simulink model "SimulinkController"  (R2026a)
settings: Solver=VariableStepAuto
libraries: cstblocks_lti x6, simulink_extras x4
settings Model: Creator=ASUS TUF  LastModifiedBy=ASUS TUF

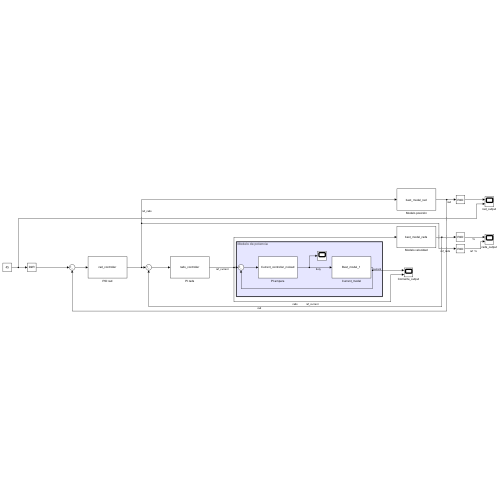
[thumbnail: Simulink's stored preview of the top-level diagram]
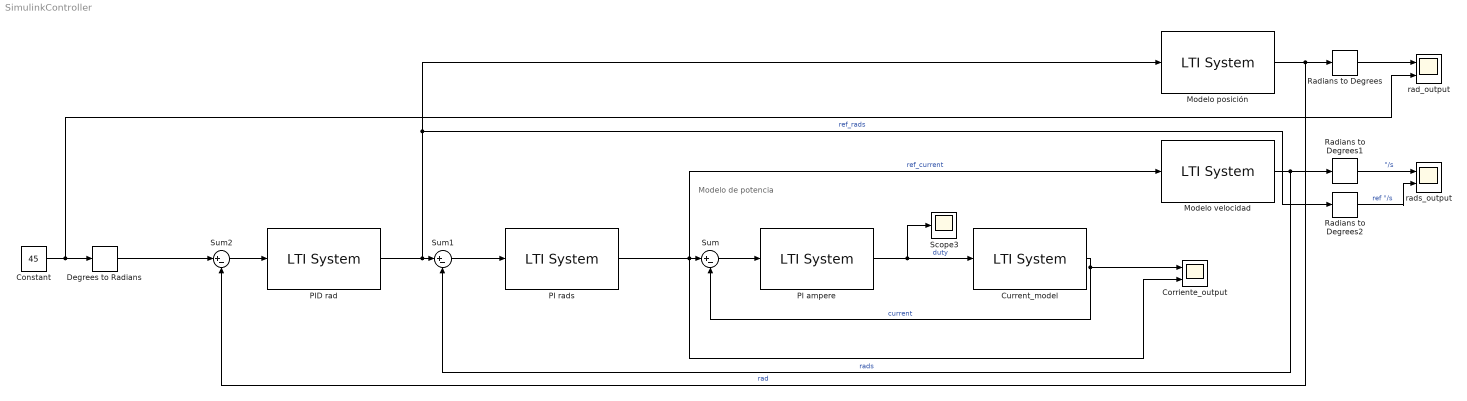
== system SimulinkController ==
  note: Modelo de potencia
  Constant : Constant  Value=45
  Corriente_output : Scope  NumInputPorts=2
      settings: ActiveDisplayYMinimum=-0.62150273899419251  ActiveDisplayYMaximum=1.3179652296290922
  Current_model : cstblocks_lti/LTI System  sys=Best_model_1  IC=[]  PadeOrder=0
      settings: LibrarySourceBlock=cstblocks/LTI System
  Degrees to Radians : simulink_extras/Transformations/Degrees to Radians
  Modelo posición : cstblocks_lti/LTI System  sys=best_model_rad  IC=[]  PadeOrder=0
      settings: LibrarySourceBlock=cstblocks/LTI System
  Modelo velocidad : cstblocks_lti/LTI System  sys=best_model_rads  IC=[]  PadeOrder=0
      settings: LibrarySourceBlock=cstblocks/LTI System
  PI ampere : cstblocks_lti/LTI System  sys=Current_controller_noload  IC=[]  PadeOrder=0
      settings: LibrarySourceBlock=cstblocks/LTI System
  PI rads : cstblocks_lti/LTI System  sys=rads_controller  IC=[]  PadeOrder=0
      settings: LibrarySourceBlock=cstblocks/LTI System
  PID rad : cstblocks_lti/LTI System  sys=rad_controller  IC=[]  PadeOrder=0
      settings: LibrarySourceBlock=cstblocks/LTI System
  Radians to Degrees : simulink_extras/Transformations/Radians to Degrees
  Radians to Degrees1 : simulink_extras/Transformations/Radians to Degrees
  Radians to Degrees2 : simulink_extras/Transformations/Radians to Degrees
  Scope3 : Scope
      settings: ActiveDisplayYMinimum=-119.11311238665843  ActiveDisplayYMaximum=302.320334328517  DataLoggingVariableName=ScopeData3
  Sum : Sum  Inputs=|+-
  Sum1 : Sum  Inputs=|+-
  Sum2 : Sum  Inputs=|+-
  rad_output : Scope  NumInputPorts=2
      settings: ActiveDisplayYMinimum=43.530744044308463  ActiveDisplayYMaximum=48.236805951806687  DataLoggingVariableName=ScopeData2
  rads_output : Scope  NumInputPorts=2
      settings: ActiveDisplayYMinimum=-55.317052883985525  ActiveDisplayYMaximum=1161.5756035421023
  wires:
  PI ampere/1 -> Scope3/1, Current_model/1  "duty"
  Sum/1 -> PI ampere/1
  Current_model/1 -> Sum/2, Corriente_output/1  "current"
  PI rads/1 -> Modelo velocidad/1, Sum/1, Corriente_output/2  "ref_current"
  Sum1/1 -> PI rads/1
  Modelo velocidad/1 -> Radians to Degrees1/1, Sum1/2  "rads"
  Modelo posición/1 -> Radians to Degrees/1, Sum2/2  "rad"
  PID rad/1 -> Radians to Degrees2/1, Modelo posición/1, Sum1/1  "ref_rads"
  Sum2/1 -> PID rad/1
  Degrees to Radians/1 -> Sum2/1
  Constant/1 -> rad_output/2, Degrees to Radians/1
  Radians to Degrees/1 -> rad_output/1
  Radians to Degrees1/1 -> rads_output/1  "°/s"
  Radians to Degrees2/1 -> rads_output/2  "ref °/s"
